simulink model "Full_Car_Model"  (R2023b)
settings: Solver=FixedStepAuto  StartTime=0.0  StopTime=t_end_sim  FixedStep=Ts_sim  RelTol=1e-3
values from neighbouring files (symbols this model uses):
  a_b_ref_sat = [ zeros(1,10) ... (first row only)    [A1_Init.m]    (also in C1_MonteCarloAnalysis.m)
  adaptive = 3    [A1_Init.m]    (also in C1_MonteCarloAnalysis.m = 1)
  data = A2_Full_car_model_parameters_4onBoard()    [A1_Init.m]    (also in C1_MonteCarloAnalysis.m)
  Ft_demand_F = [zeros(1,601) 200*ones(1,2400)]./data.R_F    [A1_Init.m]    (also in C1_MonteCarloAnalysis.m)
  Ft_demand_R = [zeros(1,(601-length(l_discr)))              200*ones(1,(2400+length(l_discr)))]./data.R_R    [A1_Init.m]    (also in C1_MonteCarloAnalysis.m)
  handmade_front = strcat(currentPath,'\Road_profiles\height_crg_files\','handmade_step_3cm_singlefunctions.crg')    [A1_Init.m]    (also in C1_MonteCarloAnalysis.m)
  handmade_mu_front = strcat(currentPath,'\Road_profiles\friction_crg_files\','handmade_fric_step_01_singlefunctions.crg')    [A1_Init.m]    (also in C1_MonteCarloAnalysis.m)
  handmade_mu_rear = handmade_mu_front    [A1_Init.m]    (also in C1_MonteCarloAnalysis.m)
  handmade_rear = handmade_front    [A1_Init.m]    (also in C1_MonteCarloAnalysis.m)
  LowLim_Q1 = -10    [A1_Init.m]    (also in C1_MonteCarloAnalysis.m)
  M = N    (= 10)    [A1_Init.m]    (also in C1_MonteCarloAnalysis.m)
  mu_distance = test_distance    [A1_Init.m]    (also in C1_MonteCarloAnalysis.m)
  mu_road = [ones(1,1001), 0.1*ones(1,2000)]    [A1_Init.m]    (also in C1_MonteCarloAnalysis.m)
  N = 10    [A1_Init.m]    (also in C1_MonteCarloAnalysis.m)
  N_iter = 3    [A1_Init.m]    (also in C1_MonteCarloAnalysis.m)
  omega_ini_F_L = x_u_dot_ini_F_L/data.R_F    [A1_Init.m]    (also in C1_MonteCarloAnalysis.m)
  omega_ini_F_R = x_u_dot_ini_R_R/data.R_F    [A1_Init.m]    (also in C1_MonteCarloAnalysis.m)
  omega_ini_R_L = x_u_dot_ini_R_L/data.R_R +2.483*1e-6    [A1_Init.m]    (also in C1_MonteCarloAnalysis.m)
  omega_ini_R_R = x_u_dot_ini_R_R/data.R_R+2.483*1e-6    [A1_Init.m]    (also in C1_MonteCarloAnalysis.m)
  passive = 2    [A1_Init.m]    (also in C1_MonteCarloAnalysis.m)
  Pitch = 0    [A1_Init.m]    (also in C1_MonteCarloAnalysis.m)
  Pitch_dot = 0    [A1_Init.m]    (also in C1_MonteCarloAnalysis.m)
  preview = 2    [A1_Init.m]    (also in C1_MonteCarloAnalysis.m)
  Q1 = 1e6    (= 1000000)    [A1_Init.m]    (also in C1_MonteCarloAnalysis.m)
  Q1_sat = 0    [A1_Init.m]    (also in C1_MonteCarloAnalysis.m)
  Q2 = 1e5    (= 100000)    [A1_Init.m]    (also in C1_MonteCarloAnalysis.m)
  QN1 = 0    [A1_Init.m]    (also in C1_MonteCarloAnalysis.m)
  QN2 = 0    [A1_Init.m]    (also in C1_MonteCarloAnalysis.m)
  R1 = 1e10    (= 10000000000)    [A1_Init.m]    (also in C1_MonteCarloAnalysis.m)
  r1_h0 = 0.99    [A1_Init.m]    (also in C1_MonteCarloAnalysis.m)
  r1_k = 1000    [A1_Init.m]    (also in C1_MonteCarloAnalysis.m)
  r1_max = 11    [A1_Init.m]    (also in C1_MonteCarloAnalysis.m)
  r1_min = -10    [A1_Init.m]    (also in C1_MonteCarloAnalysis.m)
  r2 = 2    [A1_Init.m]    (also in C1_MonteCarloAnalysis.m)
  R2 = 1e2    (= 100)    [A1_Init.m]    (also in C1_MonteCarloAnalysis.m)
  R2_rl = 2    [A1_Init.m]    (also in C1_MonteCarloAnalysis.m)
  road_profile = [zeros(1,801),ones(1,2200)*10*Step_selector]    [A1_Init.m]    (also in C1_MonteCarloAnalysis.m)
  T_distance = test_distance    [A1_Init.m]    (also in C1_MonteCarloAnalysis.m)
  T_hs_ini_F_L = 0    [A1_Init.m]    (also in C1_MonteCarloAnalysis.m)
  T_hs_ini_F_R = 0    [A1_Init.m]    (also in C1_MonteCarloAnalysis.m)
  T_hs_ini_R_L = 0    [A1_Init.m]    (also in C1_MonteCarloAnalysis.m)
  T_hs_ini_R_R = 0    [A1_Init.m]    (also in C1_MonteCarloAnalysis.m)
  test_distance = 0:0.01:30    [A1_Init.m]    (also in C1_MonteCarloAnalysis.m)
  theta_s_ini_F_L = 0    [A1_Init.m]    (also in C1_MonteCarloAnalysis.m)
  theta_s_ini_F_R = 0    [A1_Init.m]    (also in C1_MonteCarloAnalysis.m)
  theta_s_ini_R_L = 0    [A1_Init.m]    (also in C1_MonteCarloAnalysis.m)
  theta_s_ini_R_R = 0    [A1_Init.m]    (also in C1_MonteCarloAnalysis.m)
  theta_w_ini_F_L = -1.056*1e-2    (= -0.01056)    [A1_Init.m]    (also in C1_MonteCarloAnalysis.m)
  theta_w_ini_R_L = -1.056*1e-2    (= -0.01056)    [A1_Init.m]    (also in C1_MonteCarloAnalysis.m)
  Ts = 1e-3*[0 5 10 15 20 25 30 40 60 80 100]    [A1_Init.m]    (also in C1_MonteCarloAnalysis.m)
  w1_h0 = 0.0008    [A1_Init.m]    (also in C1_MonteCarloAnalysis.m)
  w1_k = 5000    [A1_Init.m]    (also in C1_MonteCarloAnalysis.m)
  w1_max = 9    [A1_Init.m]    (also in C1_MonteCarloAnalysis.m)
  w1_min = -10    [A1_Init.m]    (also in C1_MonteCarloAnalysis.m)
  w1_sat = 0.085    [A1_Init.m]    (also in C1_MonteCarloAnalysis.m)
  w2_h0 = 2    [A1_Init.m]    (also in C1_MonteCarloAnalysis.m)
  w2_inc = 0.05    [A1_Init.m]    (also in C1_MonteCarloAnalysis.m)
  w2_k = 10    [A1_Init.m]    (also in C1_MonteCarloAnalysis.m)
  w2_max = 5.3    [A1_Init.m]    (also in C1_MonteCarloAnalysis.m)
  w2_min = -10    [A1_Init.m]    (also in C1_MonteCarloAnalysis.m)
  Wmat_NMPC_init = [W(1,:) W(2,:) W(3,:) W(4,:)]    [A1_Init.m]    (also in C1_MonteCarloAnalysis.m)
  WNmat_NMPC_init = [WN(1,:) WN(2,:)]    [A1_Init.m]    (also in C1_MonteCarloAnalysis.m)
  X_0 = [z_b_dot_ini z_b_ini z_u_dot_ini_F_L z_u_ini_F_L x_b_dot_ini x_b_ini x_u_dot_ini_F_L x_u_ini_F_L          omega_ini_F_L theta_w_ini_F_L omega_ini_F_L theta_s_ini_F_L torque_ini_F_L]    [A1_Init.m]    (also in C1_MonteCarloAnalysis.m)
  x_b_dot_ini = speed_ini/3.6    (= 11.1111111111)    [A1_Init.m]    (also in C1_MonteCarloAnalysis.m)
  x_b_ini = data.b+pos_ini    [A1_Init.m]    (also in C1_MonteCarloAnalysis.m)
  x_u_dot_ini_F_L = speed_ini/3.6 - 1.125*1e-4    (= 11.1109986111)    [A1_Init.m]    (also in C1_MonteCarloAnalysis.m)
  x_u_dot_ini_F_R = speed_ini/3.6 - 1.125*1e-4    (= 11.1109986111)    [A1_Init.m]    (also in C1_MonteCarloAnalysis.m)
  x_u_dot_ini_R_L = speed_ini/3.6 - 1.125*1e-4    (= 11.1109986111)    [A1_Init.m]    (also in C1_MonteCarloAnalysis.m)
  x_u_dot_ini_R_R = speed_ini/3.6 - 1.125*1e-4    (= 11.1109986111)    [A1_Init.m]    (also in C1_MonteCarloAnalysis.m)
  x_u_ini_F_L = data.a+data.b+pos_ini    [A1_Init.m]    (also in C1_MonteCarloAnalysis.m)
  x_u_ini_F_R = data.a+data.b+pos_ini    [A1_Init.m]    (also in C1_MonteCarloAnalysis.m)
  x_u_ini_R_L = pos_ini    (= 0)    [A1_Init.m]    (also in C1_MonteCarloAnalysis.m)
  x_u_ini_R_R = pos_ini    (= 0)    [A1_Init.m]    (also in C1_MonteCarloAnalysis.m)
  z_b_dot_ini = 0    [A1_Init.m]    (also in C1_MonteCarloAnalysis.m)
  z_b_ini = 0    [A1_Init.m]    (also in C1_MonteCarloAnalysis.m)
  z_u_dot_ini_F_L = 0    [A1_Init.m]    (also in C1_MonteCarloAnalysis.m)
  z_u_dot_ini_F_R = 0    [A1_Init.m]    (also in C1_MonteCarloAnalysis.m)
  z_u_dot_ini_R_L = 0    [A1_Init.m]    (also in C1_MonteCarloAnalysis.m)
  z_u_dot_ini_R_R = 0    [A1_Init.m]    (also in C1_MonteCarloAnalysis.m)
  z_u_ini_F_L = 0    [A1_Init.m]    (also in C1_MonteCarloAnalysis.m)
  z_u_ini_F_R = 0    [A1_Init.m]    (also in C1_MonteCarloAnalysis.m)
  z_u_ini_R_L = 0    [A1_Init.m]    (also in C1_MonteCarloAnalysis.m)
  z_u_ini_R_R = 0    [A1_Init.m]    (also in C1_MonteCarloAnalysis.m)
undefined symbols (not defined in the file or in its folder): Delay_step, road_with_noise
libraries: mfswift_library x8, rllib x4, simulink x4
(part 3 of 7)

== system Full_Car_Model/CONTROLLER FRONT RIGHT/Weight matrixes ==
  x_u : Inport
  MATLAB Function : MATLAB Function  TreatAsAtomicUnit=on
  Q1 : Lookup_n-D  NumberOfTableDimensions=1  BreakpointsForDimension1=[0 1e6]  Table=[Q1 Q1]  InternalRulePriority=Speed  RndMeth=Simplest
  Q2 : Lookup_n-D  NumberOfTableDimensions=1  BreakpointsForDimension1=[0 1e6]  Table=[Q2 Q2]  InternalRulePriority=Speed  RndMeth=Simplest
  QN1 : Lookup_n-D  NumberOfTableDimensions=1  BreakpointsForDimension1=[0 1e6]  Table=[QN1 QN1]  InternalRulePriority=Speed  RndMeth=Simplest
  QN2 : Lookup_n-D  NumberOfTableDimensions=1  BreakpointsForDimension1=[0 1e6]  Table=[QN2 QN2]  InternalRulePriority=Speed  RndMeth=Simplest
  R1 : Lookup_n-D  NumberOfTableDimensions=1  BreakpointsForDimension1=[0 1e6]  Table=[R1 R1]  InternalRulePriority=Speed  RndMeth=Simplest
  R2 : Lookup_n-D  NumberOfTableDimensions=1  BreakpointsForDimension1=[0 1e6]  Table=[R2 R2]  InternalRulePriority=Speed  RndMeth=Simplest
  Scope : Scope
  Stage Cost Matrix : Outport
  Terminal Cost Matrix : Outport  Port=2
  wires:
  QN2/1 -> MATLAB Function/4(QN2)  "QN2"
  QN1/1 -> MATLAB Function/3(QN1)  "QN1"
  R2/1 -> MATLAB Function/6(R2)  "R2"
  R1/1 -> MATLAB Function/5(R1)  "R1"
  Q2/1 -> MATLAB Function/2(Q2)  "Q2"
  Q1/1 -> MATLAB Function/1(Q1)  "Q1"
  x_u/1 -> R2/1, R1/1, QN2/1, QN1/1, Q2/1, Q1/1
  MATLAB Function/2(WNmat_NMPC) -> Terminal Cost Matrix/1
  MATLAB Function/1(Wmat_NMPC) -> Stage Cost Matrix/1, Scope/1

== system Full_Car_Model/CONTROLLER REAR LEFT/RL_weights ==
  States : Inport
  Online Data : Inport  Port=2
  a_b_ref : Inport  Port=3
  Add : Sum  Inputs=+-
  Add1 : Sum  Inputs=+-
  Add2 : Sum  Inputs=+-
  Bus Selector : BusSelector  OutputSignals=Accelerations.x_b_ddot,Differentials.theta_s_dot_R_L,States.omega_R_L,States.slip_R_L,Traction_forces.Tm_R_L_req
  Control action R : Scope
  Demux : Demux  Commented=on  Outputs=3
  MATLAB Function : MATLAB Function  TreatAsAtomicUnit=on
  MATLAB Function3 : MATLAB Function  TreatAsAtomicUnit=on
  Memory1 : Memory  Commented=on  InheritSampleTime=on
  Memory2 : Memory  InheritSampleTime=on
  Memory4 : Memory  Commented=on  InheritSampleTime=on
  Memory5 : Memory  Commented=on  InheritSampleTime=on
  Mux : Mux  Commented=on  Inputs=3
  Mux6 : Mux  Inputs=5
  Policy : rllib/Policy  MATFile=blockAgentData_rear.mat  SimUsingCodegen=off
  Selector{,1..2,4..5} (5 alike) : Selector  InputPortWidth=1  IndexOptions=Select all  Indices=1  OutputSizes=1
  Subsystem2 : Subsystem
  To Workspace : ToWorkspace  VariableName=exponents_RL_RL  SaveFormat=Timeseries  SampleTime=-1
  Zero-Order Hold : ZeroOrderHold  SampleTime=0.001
  exponents : Outport
  tag scope: exp_RL_rear=global
  wires:
  Mux6/1 -> Policy/1
  Bus Selector/1 -> Add/1  "<x_b_ddot>"
  Add/1 -> Selector/1  "acc_error"
  Add1/1 -> Selector1/1  "delta_omega_error"
  Bus Selector/2 -> Add1/1  "<theta_s_dot_R_L>"
  Bus Selector/3 -> Add1/2  "<omega_R_L>"
  Bus Selector/4 -> Add2/2  "<slip_R_L>"
  Add2/1 -> Selector2/1  "slip_error"
  MATLAB Function3/1(h) -> Selector5/1  "r1"
  MATLAB Function/1(h) -> Selector4/1  "w1"
  Memory2/1 -> Zero-Order Hold/1, exponents/1, [exp_RL_rear], Control action R/1
  Selector/1 -> Mux6/1  "w1"
  Selector1/1 -> Mux6/2  "w1"
  Selector2/1 -> Mux6/3  "w1"
  Selector4/1 -> Mux6/4  "w1"
  Selector5/1 -> Mux6/5  "w1"
  States/1 -> Bus Selector/1
  a_b_ref/1 -> Add/2
  Policy/1 -> Memory2/1, Demux/1  "weights"
  Mux/1 -> ?
  Demux/1 -> Memory1/1
  Demux/3 -> Memory5/1
  Memory4/1 -> Mux/2
  Demux/2 -> Memory4/1
  Memory5/1 -> Mux/3
  Memory1/1 -> Mux/1
  Subsystem2/1(w_prev) -> MATLAB Function/1(w_prev)  "w_prev"
  Subsystem2/3(sigma_ref_act) -> Add2/1
  Subsystem2/2(mu_act_prev) -> MATLAB Function3/1(mu_prev)  "mu_act_prev"
  Online Data/1 -> Subsystem2/1(Online Data)
  Zero-Order Hold/1 -> To Workspace/1

== system Full_Car_Model/CONTROLLER REAR LEFT/ROAD PREVIEW ==
  F_t : Inport
  CAN : Inport  Port=2
  1-D Lookup Table : Lookup_n-D  NumberOfTableDimensions=1  BreakpointsForDimension1=[0.1:0.1:1]  Table=[0.005 0.01 0.016 0.02 0.025 0.03 0.04 0.05 0.055 0.06]  InternalRulePriority=Speed  RndMeth=Simplest
  1-D Lookup Table1 : Lookup_n-D  NumberOfTableDimensions=1  BreakpointsForDimension1=[0.1:0.1:1]  Table=[0.005 0.01 0.016 0.02 0.025 0.03 0.04 0.05 0.055 0.06]  InternalRulePriority=Speed  RndMeth=Simplest
  1-D Lookup Table2 : Lookup_n-D  NumberOfTableDimensions=1  BreakpointsForDimension1=mu_distance  Table=mu_road  InternalRulePriority=Speed  RndMeth=Simplest
  Bus Selector2 : BusSelector  OutputSignals=States.z_u_R_L
  Bus Selector3 : BusSelector  OutputSignals=States.x_u_R_L,States.x_u_dot_R_L,Traction_forces.Ft_F_req
  Constant : Constant
  Constant1 : Constant  Value=preview
  Constant2 : Constant
  Gain1 : Gain  Gain=data.R_R
  Multiply1 : Gain  Gain=data.R_F
  Multiply10 : Gain  Gain=1500/data.Tm_max
  Multiply12 : Gain  Gain=1500/data.Tm_max
  Multiport Switch2 : MultiPortSwitch  Inputs=2  SaturateOnIntegerOverflow=off  InputSameDT=off
  NO_ROAD_PREVIEW : MATLAB Function  TreatAsAtomicUnit=on
  Product : Product
  Product1 : Product
  ROAD PREVIEW : MATLAB Function  TreatAsAtomicUnit=on
  Time-based Road Preview : Subsystem
  To Workspace : ToWorkspace  VariableName=slip_ref_rear_sim  SaveFormat=Timeseries  SampleTime=-1
  To Workspace2 : ToWorkspace  VariableName=mu_rear_sim  SaveFormat=Timeseries  SampleTime=-1
  Online Data : Outport
  tag scope: mu_RL_LUT=global, slip_ref_R=global
  wires:
  CAN/1 -> Bus Selector2/1, Bus Selector3/1
  Multiport Switch2/1 -> Online Data/1
  Constant1/1 -> Multiport Switch2/1
  Bus Selector3/1 -> 1-D Lookup Table2/1, Time-based Road Preview/1(x_u)  "<x_u_R_L>"
  Bus Selector3/2 -> Time-based Road Preview/2(x_u_dot)  "<x_u_dot_R_L>"
  NO_ROAD_PREVIEW/1(OnlineData) -> Multiport Switch2/2  "Online Data"
  Time-based Road Preview/1(w) -> ROAD PREVIEW/1(w)
  Gain1/1 -> Multiply12/1, ROAD PREVIEW/3(Tm_req), NO_ROAD_PREVIEW/2(Tm_req)
  Bus Selector3/3 -> Product1/1  "<Ft_F_req>"
  Multiply1/1 -> Multiply10/1
  Bus Selector2/1 -> NO_ROAD_PREVIEW/1(w)  "<z_u_R_L>"
  1-D Lookup Table/1 -> ROAD PREVIEW/8(sigma_ref)
  Time-based Road Preview/2(beta_y) -> ROAD PREVIEW/2(beta_y)
  Product/1 -> NO_ROAD_PREVIEW/3(Tm_req_R2), ROAD PREVIEW/4(Tm_req_R2)
  Multiply12/1 -> Product/1
  ROAD PREVIEW/1(OnlineData) -> Multiport Switch2/3  "Online Data"
  Time-based Road Preview/3(mu_prev) -> 1-D Lookup Table/1, ROAD PREVIEW/7(mu_act)
  1-D Lookup Table2/1 -> 1-D Lookup Table1/1, NO_ROAD_PREVIEW/6(mu_act), [mu_RL_LUT], To Workspace2/1  "mu_R_L"
  1-D Lookup Table1/1 -> [slip_ref_R], To Workspace/1, NO_ROAD_PREVIEW/7(sigma_ref)
  [mu_RL_LUT] -> Product/2
  Product1/1 -> Multiply1/1
  [mu_FL_LUT] -> Product1/2
  F_t/1 -> Gain1/1
  Multiply10/1 -> ROAD PREVIEW/6(Tm_req_F_R), NO_ROAD_PREVIEW/4(Tm_req_F_L), NO_ROAD_PREVIEW/5(Tm_req_F_R), ROAD PREVIEW/5(Tm_req_F_L)

== system Full_Car_Model/CONTROLLER REAR LEFT/Reference acceleration ==
  Ft : Inport
  x_b_dot : Inport  Port=2
  Ft2 : Inport  Port=3
  2-D Lookup Table : Lookup_n-D  BreakpointsForDimension1=[0:50:350]  BreakpointsForDimension2=[0.1:0.1:1]  Table=a_b_ref_sat  InternalRulePriority=Speed  RndMeth=Simplest
      settings: InputPortMap=u0,u1
  2-D Lookup Table1 : Lookup_n-D  BreakpointsForDimension1=[0:50:350]  BreakpointsForDimension2=[0.1:0.1:1]  Table=a_b_ref_sat  InternalRulePriority=Speed  RndMeth=Simplest
      settings: InputPortMap=u0,u1
  Add : Sum
  Add1 : Sum
  Constant : Constant  Value=-Inf
  Gain : Gain  Gain=0.5
  Gain1 : Gain  Gain=0.5
  Gain2 : Gain  Gain=data.R_R
  Gain3 : Gain  Gain=data.R_F
  Saturation Dynamic : simulink/Discontinuities/Saturation Dynamic  OutMin=[]  OutMax=[]  OutDataTypeStr=Inherit: Same as second input  OutDataType=fixdt(1, 16)  OutScaling=2^-10  DoSatur=off
  a_b_ref : MATLAB Function  TreatAsAtomicUnit=on
  a_ref : Outport
  wires:
  Ft/1 -> Add/1, Gain2/1  "Ft"
  Gain2/1 -> 2-D Lookup Table/1
  Constant/1 -> Saturation Dynamic/3
  Saturation Dynamic/1 -> a_ref/1  "a_b_ref"
  x_b_dot/1 -> a_b_ref/2(vCar_k)  "x_b_dot"
  a_b_ref/1(a_b_ref) -> Saturation Dynamic/2
  Add/1 -> a_b_ref/1(Ft)
  Ft2/1 -> Gain3/1, Add/2  "Ft2"
  Add1/1 -> Saturation Dynamic/1
  Gain3/1 -> 2-D Lookup Table1/1
  [mu_RL_LUT] -> 2-D Lookup Table/2
  [mu_FL_LUT] -> 2-D Lookup Table1/2
  2-D Lookup Table1/1 -> Gain1/1
  2-D Lookup Table/1 -> Gain/1
  Gain/1 -> Add1/1
  Gain1/1 -> Add1/2

== system Full_Car_Model/CONTROLLER REAR LEFT/Rule based ==
  Online Data : Inport
  BUS : Inport  Port=2
  Flag : Subsystem
  Gain4 : Gain  Gain=data.R_R
  MATLAB Function : MATLAB Function  TreatAsAtomicUnit=on
  MATLAB Function2 : MATLAB Function  TreatAsAtomicUnit=on
  MATLAB Function3 : MATLAB Function  TreatAsAtomicUnit=on
  Min : MinMax  Inputs=2
  Mux : Mux  Inputs=3
  Product : Product
  Selector : Selector  NumberOfDimensions=2  InputPortWidth=1  IndexOptions=Index vector (dialog),Select all  Indices=1,1  OutputSizes=1,1
  Subsystem : Subsystem
  To Workspace9 : ToWorkspace  VariableName=exponents_RL_RB  SaveFormat=Timeseries  SampleTime=-1
  Zero-Order Hold : ZeroOrderHold  SampleTime=0.001
  memory : Subsystem
  exponents : Outport
  tag scope: exp_RB_rear=global
  wires:
  Min/1 -> MATLAB Function/2(mu)
  [mu_FL_LUT] -> Min/1
  MATLAB Function3/1(W) -> Mux/3  "r1"
  Subsystem/1(w_prev) -> MATLAB Function/1(w_prev)  "w_prev"
  Selector/1 -> Min/2, Product/1, MATLAB Function2/2(mu)
  Gain4/1 -> memory/1(In1)
  memory/1(Out1) -> MATLAB Function2/1(dT_req)
  [Ft_req_R] -> Product/2
  Online Data/1 -> Subsystem/1(Online Data)
  MATLAB Function2/1(W) -> Mux/2  "w2"
  MATLAB Function/1(W) -> Mux/1  "w1"
  Mux/1 -> exponents/1, [exp_RB_rear], Zero-Order Hold/1
  Zero-Order Hold/1 -> To Workspace9/1
  Product/1 -> Gain4/1
  Flag/1(Flag) -> MATLAB Function3/1(flag)
  Subsystem/2(mu_act_prev) -> Flag/2(mu_prev), MATLAB Function3/2(mu_prev), Selector/1  "mu_act_prev"
  BUS/1 -> Flag/1(Measurement data)

== system Full_Car_Model/CONTROLLER REAR LEFT/Subsystem1 ==
  exponents : Inport
  Constant : Constant  Value=R2_rl
  Constant1 : Constant  Value=0
  Demux : Demux  Outputs=3
  Exp{,1..3} (4 alike) : Math  Operator=10^u
  MATLAB Function : MATLAB Function  TreatAsAtomicUnit=on
  MATLAB Function1 : MATLAB Function  TreatAsAtomicUnit=on
  MATLAB Function2 : MATLAB Function  TreatAsAtomicUnit=on
  Min : MinMax  Inputs=2
  stage cost matrix : Outport
  terminal cost matrix : Outport  Port=2
  wires:
  MATLAB Function/1(Wmat_NMPC) -> stage cost matrix/1
  MATLAB Function1/1(WNmat_NMPC) -> terminal cost matrix/1
  exponents/1 -> Demux/1
  Demux/1 -> MATLAB Function2/1(Q1)
  Demux/2 -> Exp1/1
  Demux/3 -> Exp2/1
  Exp/1 -> MATLAB Function/1(Q1)
  Exp1/1 -> MATLAB Function/2(Q2)
  Exp2/1 -> MATLAB Function/3(R1)
  Constant/1 -> Exp3/1
  Exp3/1 -> MATLAB Function/4(R2)
  Constant1/1 -> MATLAB Function1/2(QN2), MATLAB Function1/1(QN1)
  [mu_FL_LUT] -> Min/1
  [mu_RL_LUT] -> Min/2
  Min/1 -> MATLAB Function2/2(mu)
  MATLAB Function2/1(Q1_out) -> Exp/1

== system Full_Car_Model/CONTROLLER REAR LEFT/Subsystem2 ==
  exponents : Inport
  Constant : Constant  Value=r2
  Constant1 : Constant  Value=0
  Demux : Demux  Outputs=3
  Exp{,1..4} (5 alike) : Math  Operator=10^u
  MATLAB Function : MATLAB Function  TreatAsAtomicUnit=on
  MATLAB Function1 : MATLAB Function  TreatAsAtomicUnit=on
  stage cost matrix : Outport
  terminal cost matrix : Outport  Port=2
  wires:
  MATLAB Function/1(Wmat_NMPC) -> stage cost matrix/1
  MATLAB Function1/1(WNmat_NMPC) -> terminal cost matrix/1
  exponents/1 -> Demux/1
  Demux/1 -> Exp/1
  Demux/2 -> Exp1/1
  Demux/3 -> Exp2/1
  Exp/1 -> MATLAB Function/1(Q1)
  Exp1/1 -> MATLAB Function/2(Q2)
  Exp2/1 -> MATLAB Function/3(R1)
  Constant/1 -> Exp3/1
  Exp3/1 -> MATLAB Function/4(R2)
  Constant1/1 -> Exp4/1
  Exp4/1 -> MATLAB Function1/2(QN2), MATLAB Function1/1(QN1)

== system Full_Car_Model/CONTROLLER REAR LEFT/Weight matrixes ==
  x_u : Inport
  MATLAB Function : MATLAB Function  TreatAsAtomicUnit=on
  Q1 : Lookup_n-D  NumberOfTableDimensions=1  BreakpointsForDimension1=[0 1e6]  Table=[Q1 Q1]  InternalRulePriority=Speed  RndMeth=Simplest
  Q2 : Lookup_n-D  NumberOfTableDimensions=1  BreakpointsForDimension1=[0 1e6]  Table=[Q2 Q2]  InternalRulePriority=Speed  RndMeth=Simplest
  QN1 : Lookup_n-D  NumberOfTableDimensions=1  BreakpointsForDimension1=[0 1e6]  Table=[QN1 QN1]  InternalRulePriority=Speed  RndMeth=Simplest
  QN2 : Lookup_n-D  NumberOfTableDimensions=1  BreakpointsForDimension1=[0 1e6]  Table=[QN2 QN2]  InternalRulePriority=Speed  RndMeth=Simplest
  R1 : Lookup_n-D  NumberOfTableDimensions=1  BreakpointsForDimension1=[0 1e6]  Table=[R1 R1]  InternalRulePriority=Speed  RndMeth=Simplest
  R2 : Lookup_n-D  NumberOfTableDimensions=1  BreakpointsForDimension1=[0 1e6]  Table=[R2 R2]  InternalRulePriority=Speed  RndMeth=Simplest
  Scope : Scope
  Stage Cost Matrix : Outport
  Terminal Cost Matrix : Outport  Port=2
  wires:
  QN2/1 -> MATLAB Function/4(QN2)  "QN2"
  QN1/1 -> MATLAB Function/3(QN1)  "QN1"
  R2/1 -> MATLAB Function/6(R2)  "R2"
  R1/1 -> MATLAB Function/5(R1)  "R1"
  Q2/1 -> MATLAB Function/2(Q2)  "Q2"
  Q1/1 -> MATLAB Function/1(Q1)  "Q1"
  x_u/1 -> R2/1, R1/1, QN2/1, QN1/1, Q2/1, Q1/1
  MATLAB Function/2(WNmat_NMPC) -> Terminal Cost Matrix/1
  MATLAB Function/1(Wmat_NMPC) -> Stage Cost Matrix/1, Scope/1

== system Full_Car_Model/CONTROLLER REAR RIGHT/RL_weights ==
  States : Inport
  Online Data : Inport  Port=2
  a_b_ref : Inport  Port=3
  Add : Sum  Inputs=+-
  Add1 : Sum  Inputs=+-
  Add2 : Sum  Inputs=+-
  Bus Selector : BusSelector  OutputSignals=Accelerations.x_b_ddot,Differentials.theta_s_dot_R_R,States.omega_R_R,States.slip_R_R
  Control action : Scope
  Demux : Demux  Commented=on  Outputs=3
  MATLAB Function : MATLAB Function  TreatAsAtomicUnit=on
  MATLAB Function3 : MATLAB Function  TreatAsAtomicUnit=on
  Memory1 : Memory  Commented=on  InheritSampleTime=on
  Memory2 : Memory  InheritSampleTime=on
  Memory4 : Memory  Commented=on  InheritSampleTime=on
  Memory5 : Memory  Commented=on  InheritSampleTime=on
  Mux : Mux  Commented=on  Inputs=3
  Mux6 : Mux  Inputs=5
  Policy : rllib/Policy  MATFile=blockAgentData_rear.mat  SimUsingCodegen=off
  Selector{,1..2,4..5} (5 alike) : Selector  InputPortWidth=1  IndexOptions=Select all  Indices=1  OutputSizes=1
  Subsystem2 : Subsystem
  exponents : Outport
  wires:
  Mux6/1 -> Policy/1
  Bus Selector/1 -> Add/1  "<x_b_ddot>"
  Add/1 -> Selector/1  "acc_error"
  Add1/1 -> Selector1/1  "delta_omega_error"
  Bus Selector/2 -> Add1/1  "<theta_s_dot_R_R>"
  Bus Selector/3 -> Add1/2  "<omega_R_R>"
  Bus Selector/4 -> Add2/2  "<slip_R_R>"
  Add2/1 -> Selector2/1  "slip_error"
  Memory2/1 -> Control action/1, exponents/1
  Selector/1 -> Mux6/1  "w1"
  Selector1/1 -> Mux6/2  "w1"
  Selector2/1 -> Mux6/3  "w1"
  Selector4/1 -> Mux6/4  "w1"
  Selector5/1 -> Mux6/5  "w1"
  States/1 -> Bus Selector/1
  a_b_ref/1 -> Add/2
  Online Data/1 -> Subsystem2/1(Online Data)
  Mux/1 -> ?
  Demux/1 -> Memory1/1
  Policy/1 -> Memory2/1, Demux/1  "weights"
  Demux/3 -> Memory5/1
  Memory4/1 -> Mux/2
  Demux/2 -> Memory4/1
  Memory5/1 -> Mux/3
  Memory1/1 -> Mux/1
  Subsystem2/1(w_prev) -> MATLAB Function/1(w_prev)  "w_prev"
  Subsystem2/3(sigma_ref_act) -> Add2/1
  Subsystem2/2(mu_act_prev) -> MATLAB Function3/1(mu_prev)  "mu_act_prev"
  MATLAB Function/1(h) -> Selector4/1  "w1"
  MATLAB Function3/1(h) -> Selector5/1  "r1"

== system Full_Car_Model/CONTROLLER REAR RIGHT/ROAD PREVIEW ==
  F_t : Inport
  CAN : Inport  Port=2
  1-D Lookup Table : Lookup_n-D  NumberOfTableDimensions=1  BreakpointsForDimension1=[0.1:0.1:1]  Table=[0.005 0.01 0.016 0.02 0.025 0.03 0.04 0.05 0.055 0.06]  InternalRulePriority=Speed  RndMeth=Simplest
  1-D Lookup Table1 : Lookup_n-D  NumberOfTableDimensions=1  BreakpointsForDimension1=[0.1:0.1:1]  Table=[0.005 0.01 0.016 0.02 0.025 0.03 0.04 0.05 0.055 0.06]  InternalRulePriority=Speed  RndMeth=Simplest
  1-D Lookup Table2 : Lookup_n-D  NumberOfTableDimensions=1  BreakpointsForDimension1=mu_distance  Table=mu_road  InternalRulePriority=Speed  RndMeth=Simplest
  Bus Selector2 : BusSelector  OutputSignals=States.z_u_R_R
  Bus Selector3 : BusSelector  OutputSignals=States.x_u_R_R,States.x_u_dot_R_R,Traction_forces.Ft_F_req
  Constant : Constant
  Constant1 : Constant  Value=preview
  Constant2 : Constant
  Gain3 : Gain  Gain=data.R_R
  Multiply4 : Gain  Gain=data.R_F
  Multiply5 : Gain  Gain=1500/data.Tm_max
  Multiply6 : Gain  Gain=1500/data.Tm_max
  Multiport Switch2 : MultiPortSwitch  Inputs=2  SaturateOnIntegerOverflow=off  InputSameDT=off
  NO_ROAD_PREVIEW : MATLAB Function  TreatAsAtomicUnit=on
  Product2 : Product
  Product3 : Product
  ROAD PREVIEW : MATLAB Function  TreatAsAtomicUnit=on
  Time-based Road Preview : Subsystem
  Online Data : Outport
  tag scope: mu_RR_LUT=global
  wires:
  1-D Lookup Table1/1 -> NO_ROAD_PREVIEW/7(sigma_ref)
  Time-based Road Preview/3(mu_prev) -> 1-D Lookup Table/1, ROAD PREVIEW/7(mu_act)
  Product2/1 -> NO_ROAD_PREVIEW/3(Tm_req_R2), ROAD PREVIEW/4(Tm_req_R2)
  CAN/1 -> Bus Selector2/1, Bus Selector3/1
  Multiport Switch2/1 -> Online Data/1
  Bus Selector2/1 -> NO_ROAD_PREVIEW/1(w)  "<z_u_R_R>"
  Time-based Road Preview/1(w) -> ROAD PREVIEW/1(w)
  Time-based Road Preview/2(beta_y) -> ROAD PREVIEW/2(beta_y)
  Multiply5/1 -> ROAD PREVIEW/6(Tm_req_F_R), NO_ROAD_PREVIEW/4(Tm_req_F_L), NO_ROAD_PREVIEW/5(Tm_req_F_R), ROAD PREVIEW/5(Tm_req_F_L)
  1-D Lookup Table/1 -> ROAD PREVIEW/8(sigma_ref)
  ROAD PREVIEW/1(OnlineData) -> Multiport Switch2/3  "Online Data"
  Bus Selector3/1 -> 1-D Lookup Table2/1, Time-based Road Preview/1(x_u)  "<x_u_R_R>"
  Bus Selector3/2 -> Time-based Road Preview/2(x_u_dot)  "<x_u_dot_R_R>"
  NO_ROAD_PREVIEW/1(OnlineData) -> Multiport Switch2/2  "Online Data"
  Constant1/1 -> Multiport Switch2/1
  1-D Lookup Table2/1 -> [mu_RR_LUT], 1-D Lookup Table1/1, NO_ROAD_PREVIEW/6(mu_act)  "mu_R_R"
  Gain3/1 -> ROAD PREVIEW/3(Tm_req), Multiply6/1, NO_ROAD_PREVIEW/2(Tm_req)
  Bus Selector3/3 -> Product3/1  "<Ft_F_req>"
  [mu_RL_LUT] -> Product2/2
  [mu_FL_LUT] -> Product3/2
  Multiply6/1 -> Product2/1
  Product3/1 -> Multiply4/1
  F_t/1 -> Gain3/1
  Multiply4/1 -> Multiply5/1

== system Full_Car_Model/CONTROLLER REAR RIGHT/Reference acceleration ==
  Ft : Inport
  x_b_dot : Inport  Port=2
  Ft2 : Inport  Port=3
  2-D Lookup Table : Lookup_n-D  BreakpointsForDimension1=[0:50:350]  BreakpointsForDimension2=[0.1:0.1:1]  Table=a_b_ref_sat  InternalRulePriority=Speed  RndMeth=Simplest
      settings: InputPortMap=u0,u1
  2-D Lookup Table1 : Lookup_n-D  BreakpointsForDimension1=[0:50:350]  BreakpointsForDimension2=[0.1:0.1:1]  Table=a_b_ref_sat  InternalRulePriority=Speed  RndMeth=Simplest
      settings: InputPortMap=u0,u1
  Add : Sum
  Add1 : Sum
  Constant : Constant  Value=-Inf
  Gain : Gain  Gain=0.5
  Gain1 : Gain  Gain=0.5
  Gain2 : Gain  Gain=data.R_R
  Gain3 : Gain  Gain=data.R_F
  Saturation Dynamic : simulink/Discontinuities/Saturation Dynamic  OutMin=[]  OutMax=[]  OutDataTypeStr=Inherit: Same as second input  OutDataType=fixdt(1, 16)  OutScaling=2^-10  DoSatur=off
  a_b_ref : MATLAB Function  TreatAsAtomicUnit=on
  a_ref : Outport
  wires:
  Ft/1 -> Add/1, Gain2/1  "Ft"
  Gain2/1 -> 2-D Lookup Table/1
  Constant/1 -> Saturation Dynamic/3
  Saturation Dynamic/1 -> a_ref/1  "a_b_ref"
  x_b_dot/1 -> a_b_ref/2(vCar_k)  "x_b_dot"
  a_b_ref/1(a_b_ref) -> Saturation Dynamic/2
  Add/1 -> a_b_ref/1(Ft)
  Ft2/1 -> Gain3/1, Add/2  "Ft2"
  Add1/1 -> Saturation Dynamic/1
  Gain3/1 -> 2-D Lookup Table1/1
  [mu_RL_LUT] -> 2-D Lookup Table/2
  [mu_FL_LUT] -> 2-D Lookup Table1/2
  2-D Lookup Table1/1 -> Gain1/1
  2-D Lookup Table/1 -> Gain/1
  Gain/1 -> Add1/1
  Gain1/1 -> Add1/2

== system Full_Car_Model/CONTROLLER REAR RIGHT/Rule based ==
  Online Data : Inport
  BUS : Inport  Port=2
  Flag : Subsystem
  Gain4 : Gain  Gain=data.R_R
  MATLAB Function : MATLAB Function  TreatAsAtomicUnit=on
  MATLAB Function2 : MATLAB Function  TreatAsAtomicUnit=on
  MATLAB Function3 : MATLAB Function  TreatAsAtomicUnit=on
  Min : MinMax  Inputs=2
  Mux : Mux  Inputs=3
  Product : Product
  Selector : Selector  NumberOfDimensions=2  InputPortWidth=1  IndexOptions=Index vector (dialog),Select all  Indices=1,1  OutputSizes=1,1
  Subsystem : Subsystem
  memory : Subsystem
  exponents : Outport
  wires:
  Min/1 -> MATLAB Function/2(mu)
  [mu_FL_LUT] -> Min/1
  MATLAB Function3/1(W) -> Mux/3  "r1"
  Subsystem/1(w_prev) -> MATLAB Function/1(w_prev)  "w_prev"
  Selector/1 -> Min/2, Product/1, MATLAB Function2/2(mu)
  Gain4/1 -> memory/1(In1)
  memory/1(Out1) -> MATLAB Function2/1(dT_req)
  [Ft_req_R] -> Product/2
  Online Data/1 -> Subsystem/1(Online Data)
  MATLAB Function2/1(W) -> Mux/2  "w2"
  MATLAB Function/1(W) -> Mux/1  "w1"
  Mux/1 -> exponents/1
  Product/1 -> Gain4/1
  Subsystem/2(mu_act_prev) -> Flag/2(mu_prev), MATLAB Function3/2(mu_prev), Selector/1  "mu_act_prev"
  Flag/1(Flag) -> MATLAB Function3/1(flag)
  BUS/1 -> Flag/1(Measurement data)

== system Full_Car_Model/CONTROLLER REAR RIGHT/Subsystem1 ==
  exponents : Inport
  Constant : Constant  Value=R2_rl
  Constant1 : Constant  Value=0
  Demux : Demux  Outputs=3
  Exp{,1..3} (4 alike) : Math  Operator=10^u
  MATLAB Function : MATLAB Function  TreatAsAtomicUnit=on
  MATLAB Function1 : MATLAB Function  TreatAsAtomicUnit=on
  MATLAB Function2 : MATLAB Function  TreatAsAtomicUnit=on
  Min : MinMax  Inputs=2
  stage cost matrix : Outport
  terminal cost matrix : Outport  Port=2
  wires:
  MATLAB Function/1(Wmat_NMPC) -> stage cost matrix/1
  MATLAB Function1/1(WNmat_NMPC) -> terminal cost matrix/1
  exponents/1 -> Demux/1
  Demux/1 -> MATLAB Function2/1(Q1)
  Demux/2 -> Exp1/1
  Demux/3 -> Exp2/1
  Exp/1 -> MATLAB Function/1(Q1)
  Exp1/1 -> MATLAB Function/2(Q2)
  Exp2/1 -> MATLAB Function/3(R1)
  Constant/1 -> Exp3/1
  Exp3/1 -> MATLAB Function/4(R2)
  Constant1/1 -> MATLAB Function1/2(QN2), MATLAB Function1/1(QN1)
  [mu_FL_LUT] -> Min/1
  [mu_RL_LUT] -> Min/2
  Min/1 -> MATLAB Function2/2(mu)
  MATLAB Function2/1(Q1_out) -> Exp/1

== system Full_Car_Model/CONTROLLER REAR RIGHT/Subsystem2 ==
  exponents : Inport
  Constant : Constant  Value=r2
  Constant1 : Constant  Value=0
  Demux : Demux  Outputs=3
  Exp{,1..4} (5 alike) : Math  Operator=10^u
  MATLAB Function : MATLAB Function  TreatAsAtomicUnit=on
  MATLAB Function1 : MATLAB Function  TreatAsAtomicUnit=on
  stage cost matrix : Outport
  terminal cost matrix : Outport  Port=2
  wires:
  MATLAB Function/1(Wmat_NMPC) -> stage cost matrix/1
  MATLAB Function1/1(WNmat_NMPC) -> terminal cost matrix/1
  exponents/1 -> Demux/1
  Demux/1 -> Exp/1
  Demux/2 -> Exp1/1
  Demux/3 -> Exp2/1
  Exp/1 -> MATLAB Function/1(Q1)
  Exp1/1 -> MATLAB Function/2(Q2)
  Exp2/1 -> MATLAB Function/3(R1)
  Constant/1 -> Exp3/1
  Exp3/1 -> MATLAB Function/4(R2)
  Constant1/1 -> Exp4/1
  Exp4/1 -> MATLAB Function1/2(QN2), MATLAB Function1/1(QN1)

== system Full_Car_Model/CONTROLLER REAR RIGHT/Weight matrixes ==
  x_u : Inport
  MATLAB Function : MATLAB Function  TreatAsAtomicUnit=on
  Q1 : Lookup_n-D  NumberOfTableDimensions=1  BreakpointsForDimension1=[0 1e6]  Table=[Q1 Q1]  InternalRulePriority=Speed  RndMeth=Simplest
  Q2 : Lookup_n-D  NumberOfTableDimensions=1  BreakpointsForDimension1=[0 1e6]  Table=[Q2 Q2]  InternalRulePriority=Speed  RndMeth=Simplest
  QN1 : Lookup_n-D  NumberOfTableDimensions=1  BreakpointsForDimension1=[0 1e6]  Table=[QN1 QN1]  InternalRulePriority=Speed  RndMeth=Simplest
  QN2 : Lookup_n-D  NumberOfTableDimensions=1  BreakpointsForDimension1=[0 1e6]  Table=[QN2 QN2]  InternalRulePriority=Speed  RndMeth=Simplest
  R1 : Lookup_n-D  NumberOfTableDimensions=1  BreakpointsForDimension1=[0 1e6]  Table=[R1 R1]  InternalRulePriority=Speed  RndMeth=Simplest
  R2 : Lookup_n-D  NumberOfTableDimensions=1  BreakpointsForDimension1=[0 1e6]  Table=[R2 R2]  InternalRulePriority=Speed  RndMeth=Simplest
  Scope : Scope
  Stage Cost Matrix : Outport
  Terminal Cost Matrix : Outport  Port=2
  wires:
  QN2/1 -> MATLAB Function/4(QN2)  "QN2"
  QN1/1 -> MATLAB Function/3(QN1)  "QN1"
  R2/1 -> MATLAB Function/6(R2)  "R2"
  R1/1 -> MATLAB Function/5(R1)  "R1"
  Q2/1 -> MATLAB Function/2(Q2)  "Q2"
  Q1/1 -> MATLAB Function/1(Q1)  "Q1"
  x_u/1 -> R2/1, R1/1, QN2/1, QN1/1, Q2/1, Q1/1
  MATLAB Function/2(WNmat_NMPC) -> Terminal Cost Matrix/1
  MATLAB Function/1(Wmat_NMPC) -> Stage Cost Matrix/1, Scope/1

== system Full_Car_Model/NMPC Internal model FL/Time-based Road Preview ==
  x_u : Inport
  Delay1 : Delay  Commented=on  DelayLength=Delay_step
  Gain1 : Gain  Gain=1e-3
  Goto5 : Goto  Commented=on  GotoTag=beta_y_env_F_L  TagVisibility=global
  Goto6 : Goto  Commented=on  GotoTag=w_env_F_L  TagVisibility=global
  MATLAB Function1 : MATLAB Function  TreatAsAtomicUnit=on
  MATLAB Function4 : MATLAB Function  TreatAsAtomicUnit=on
  MATLAB Function5 : MATLAB Function  TreatAsAtomicUnit=on
  Scope : Scope
  Z_road with noise2 : Lookup_n-D  Commented=on  NumberOfTableDimensions=1  BreakpointsForDimension1=test_distance  Table=road_with_noise  InterpMethod=Flat  InternalRulePriority=Speed  RndMeth=Simplest
  Z_road1 : Lookup_n-D  NumberOfTableDimensions=1  BreakpointsForDimension1=test_distance  Table=road_profile  InterpMethod=Flat  InternalRulePriority=Speed  RndMeth=Simplest
  w : Outport
  beta_y : Outport  Port=2
  wires:
  x_u/1 -> MATLAB Function5/1(X)
  MATLAB Function5/1(x_road) -> Z_road1/1
  Z_road1/1 -> Gain1/1
  MATLAB Function4/2(beta_y) -> Goto5/1, beta_y/1
  MATLAB Function1/1(Z_ef) -> MATLAB Function4/1(Z_ef)
  MATLAB Function1/2(Z_er) -> MATLAB Function4/2(Z_er)
  MATLAB Function4/1(w) -> Scope/1, w/1, Goto6/1  "w"
  Gain1/1 -> MATLAB Function1/1(z_road)

== system Full_Car_Model/PLANT MODEL WITH MF-SWIFT/4 ON-BOARD POWERTRAIN - FRONT ==
  T_m_L : Inport
  T_m_R : Inport  Port=2
  theta_w_L : Inport  Port=3
  omega_w_L : Inport  Port=4
  theta_w_R : Inport  Port=5
  omega_w_R : Inport  Port=6
  DIFFERENTIAL_L : Subsystem
  DIFFERENTIAL_R : Subsystem
  Integrator1 : Integrator  InitialCondition=theta_s_ini_F_L
  Integrator2 : Integrator  InitialCondition=omega_ini_F_L
  Integrator3 : Integrator  InitialCondition=theta_s_ini_F_R
  Integrator6 : Integrator  InitialCondition=omega_ini_F_R
  LEFT HALF SHAFT TORQUES WITH BACKLASH : Subsystem
  Memory : Memory  InitialCondition=T_hs_ini_F_L
  Memory1 : Memory  InitialCondition=T_hs_ini_F_R
  RIGHT HALF SHAFT TORQUES WITH BACKLASH : Subsystem
  SHAFT EQUATIONS : MATLAB Function  TreatAsAtomicUnit=on
  To Workspace : ToWorkspace  VariableName=Tm_FL_sim  SaveFormat=Timeseries  SampleTime=-1
  To Workspace1 : ToWorkspace  VariableName=Tm_FR_sim  SaveFormat=Timeseries  SampleTime=-1
  T_hs_L : Outport
  T_hs_R : Outport  Port=2
  tag scope: Tm_F_L=global, Tm_F_R=global, theta_s_F_L=global, theta_s_F_R=global, theta_s_ddot_F_L=global, theta_s_ddot_F_R=global, theta_s_dot_F_L=global, theta_s_dot_F_R=global
  wires:
  Integrator6/1 -> [theta_s_dot_F_R], Integrator3/1, RIGHT HALF SHAFT TORQUES WITH BACKLASH/1(omega_s)  "theta_s_dot_R"
  Integrator2/1 -> [theta_s_dot_F_L], Integrator1/1, LEFT HALF SHAFT TORQUES WITH BACKLASH/1(omega_s)  "theta_s_dot_L"
  Memory1/1 -> SHAFT EQUATIONS/4(T_hs_R)
  Integrator3/1 -> [theta_s_F_R], RIGHT HALF SHAFT TORQUES WITH BACKLASH/2(theta_s)  "theta_s_R"
  theta_w_R/1 -> RIGHT HALF SHAFT TORQUES WITH BACKLASH/3(theta_w)
  omega_w_L/1 -> LEFT HALF SHAFT TORQUES WITH BACKLASH/4(omega_w)
  omega_w_R/1 -> RIGHT HALF SHAFT TORQUES WITH BACKLASH/4(omega_w)
  RIGHT HALF SHAFT TORQUES WITH BACKLASH/1(T_hs) -> T_hs_R/1, Memory1/1  "T_hs_R"
  DIFFERENTIAL_L/1(T_t) -> SHAFT EQUATIONS/1(T_t_L)
  theta_w_L/1 -> LEFT HALF SHAFT TORQUES WITH BACKLASH/3(theta_w)
  Integrator1/1 -> [theta_s_F_L], LEFT HALF SHAFT TORQUES WITH BACKLASH/2(theta_s)  "theta_s_L"
  LEFT HALF SHAFT TORQUES WITH BACKLASH/1(T_hs) -> Memory/1, T_hs_L/1  "T_hs_L"
  Memory/1 -> SHAFT EQUATIONS/2(T_hs_L)
  DIFFERENTIAL_R/1(T_t) -> SHAFT EQUATIONS/3(T_t_R)
  T_m_R/1 -> [Tm_F_R], To Workspace1/1, DIFFERENTIAL_R/1(T_dm)
  T_m_L/1 -> DIFFERENTIAL_L/1(T_dm), [Tm_F_L], To Workspace/1
  SHAFT EQUATIONS/2(theta_s_ddot_R) -> [theta_s_ddot_F_R], Integrator6/1
  SHAFT EQUATIONS/1(theta_s_ddot_L) -> [theta_s_ddot_F_L], Integrator2/1

== system Full_Car_Model/PLANT MODEL WITH MF-SWIFT/4 ON-BOARD POWERTRAIN - REAR ==
  T_m_L : Inport
  T_m_R : Inport  Port=2
  theta_w_L : Inport  Port=3
  omega_w_L : Inport  Port=4
  theta_w_R : Inport  Port=5
  omega_w_R : Inport  Port=6
  DIFFERENTIAL_L : Subsystem
  DIFFERENTIAL_R : Subsystem
  Integrator1 : Integrator  InitialCondition=theta_s_ini_R_L
  Integrator3 : Integrator  InitialCondition=theta_s_ini_R_R
  Integrator4 : Integrator  InitialCondition=omega_ini_R_L
  Integrator5 : Integrator  InitialCondition=omega_ini_R_R
  LEFT HALF SHAFT TORQUES WITH BACKLASH : Subsystem
  Memory : Memory  InitialCondition=T_hs_ini_R_L
  Memory1 : Memory  InitialCondition=T_hs_ini_R_R
  OPEN DIFFERENTIAL EQUATIONS : MATLAB Function  TreatAsAtomicUnit=on
  RIGHT HALF SHAFT TORQUES WITH BACKLASH : Subsystem
  To Workspace : ToWorkspace  VariableName=Tm_RL_sim  SaveFormat=Timeseries  SampleTime=-1
  To Workspace1 : ToWorkspace  VariableName=Tm_RR_sim  SaveFormat=Timeseries  SampleTime=-1
  T_hs_L : Outport
  T_hs_R : Outport  Port=2
  tag scope: Tm_R_L=global, Tm_R_R=global, theta_s_R_L=global, theta_s_R_R=global, theta_s_ddot_R_L=global, theta_s_ddot_R_R=global, theta_s_dot_R_L=global, theta_s_dot_R_R=global
  wires:
  Integrator5/1 -> [theta_s_dot_R_R], RIGHT HALF SHAFT TORQUES WITH BACKLASH/1(omega_s), Integrator3/1  "theta_s_dot_R"
  Integrator4/1 -> [theta_s_dot_R_L], Integrator1/1, LEFT HALF SHAFT TORQUES WITH BACKLASH/1(omega_s)  "theta_s_dot_L"
  Memory1/1 -> OPEN DIFFERENTIAL EQUATIONS/4(T_hs_R)
  Integrator3/1 -> [theta_s_R_R], RIGHT HALF SHAFT TORQUES WITH BACKLASH/2(theta_s)  "theta_s_R"
  theta_w_R/1 -> RIGHT HALF SHAFT TORQUES WITH BACKLASH/3(theta_w)
  omega_w_L/1 -> LEFT HALF SHAFT TORQUES WITH BACKLASH/4(omega_w)
  omega_w_R/1 -> RIGHT HALF SHAFT TORQUES WITH BACKLASH/4(omega_w)
  DIFFERENTIAL_L/1(T_t) -> OPEN DIFFERENTIAL EQUATIONS/1(T_t_L)
  theta_w_L/1 -> LEFT HALF SHAFT TORQUES WITH BACKLASH/3(theta_w)
  Integrator1/1 -> [theta_s_R_L], LEFT HALF SHAFT TORQUES WITH BACKLASH/2(theta_s)  "theta_s_L"
  Memory/1 -> OPEN DIFFERENTIAL EQUATIONS/2(T_hs_L)
  LEFT HALF SHAFT TORQUES WITH BACKLASH/1(T_hs) -> Memory/1, T_hs_L/1  "T_hs_L"
  RIGHT HALF SHAFT TORQUES WITH BACKLASH/1(T_hs) -> T_hs_R/1, Memory1/1  "T_hs_R"
  DIFFERENTIAL_R/1(T_t) -> OPEN DIFFERENTIAL EQUATIONS/3(T_t_R)
  OPEN DIFFERENTIAL EQUATIONS/1(theta_s_ddot_L) -> [theta_s_ddot_R_L], Integrator4/1
  T_m_R/1 -> [Tm_R_R], To Workspace1/1, DIFFERENTIAL_R/1(T_dm)
  T_m_L/1 -> [Tm_R_L], To Workspace/1, DIFFERENTIAL_L/1(T_dm)
  OPEN DIFFERENTIAL EQUATIONS/2(theta_s_ddot_R) -> Integrator5/1, [theta_s_ddot_R_R]

== system Full_Car_Model/PLANT MODEL WITH MF-SWIFT/FRONT LEFT WHEEL ==
  note: Front rotational balance
  Tt_F_L : Inport
  BUS : Inport  Port=2
  Add : Sum
  Bus Creator : BusCreator  Inputs=3
  Bus Selector : BusSelector  OutputSignals=vertical_deflection,effective_rolling_radius,eff_plane_height,eff_plane_angle,Fx,longitudinal_slip,effective_rolling_radius,mu_x
  Clock : Clock
  Constant2 : Constant
  Demux : Demux  Outputs=2
  Gain : Gain  Gain=1/(data.I_y_F)
  Integrate velocity : Integrator  InitialCondition=theta_w_ini_F_L
  Integrate wheel acceleration : Integrator  InitialCondition=omega_ini_F_L
  MF-Swift : mfswift_library/MF-Swift  Tag=STI tyre  idtyre=3  tpfname=tir_name_L  rdfname=[handmade_front,';',handmade_mu_front];  road_mode=(2xxxx) opencrg  side_mode=(x3xxx) symmetric  cnt_mode=(xx5xx) enveloping  dyn_mode=(xxx3x) rigid-ring  mf_mode=(xxxx1) longitudinal  tv_model=Disabled  overwrite=off  use_mode=ISWITCH  internal_solver=off  enable_rr_init=on  optional_input=''  override_typarr=off  disp_debug=off
  Scope : Scope
  "Select Fz, wheel" : Selector  InputPortWidth=3  IndexOptions=Index vector (dialog)  Indices=[1 3]  OutputSizes=[(-2)]
  Select My,wheel : Selector  InputPortWidth=3  IndexOptions=Index vector (dialog)  Indices=2  OutputSizes=[(-2)]
  Subsystem : Subsystem
  Subsystem1 : Subsystem
  Subsystem6 : Subsystem
  Terminator{1..4,12} (5 alike) : Terminator
  To Workspace2 : ToWorkspace  VariableName=force_F_L  SampleTime=-1
  To Workspace3 : ToWorkspace  VariableName=torque_F_L  SampleTime=-1
  local2global : mfswift_library/local2global  Tag=local2global  init_pos=[data.a+data.b 0 (0.3833 - 0.5*data.m_total*9.81*data.b/data.L/data.k_t_F)]  init_angle=[0 0 0]
  Fx_F_L : Outport  VectorParamsAs1DForOutWhenUnconnected=off
  Fz_F_L_tot : Outport  Port=2  VectorParamsAs1DForOutWhenUnconnected=off
  Rotational_F_L : Outport  Port=3  VectorParamsAs1DForOutWhenUnconnected=off
  Slip_F_L : Outport  Port=4  VectorParamsAs1DForOutWhenUnconnected=off
  tag scope: mu_swift_F_L=global, w_swift_F_L=global
  wires:
  Bus Selector/8 -> [mu_swift_F_L], Scope/1  "<mu_x>"
  Bus Creator/1 -> Rotational_F_L/1
  Bus Selector/7 -> Terminator1/1  "<effective_rolling_radius>"
  Bus Selector/6 -> Slip_F_L/1  "<longitudinal_slip>"
  Bus Selector/5 -> Terminator3/1  "<Fx>"
  Bus Selector/2 -> Terminator2/1  "<effective_rolling_radius>"
  Bus Selector/1 -> Terminator12/1  "<vertical_deflection>"
  Bus Selector/3 -> [w_swift_F_L]  "<eff_plane_height>"
  Bus Selector/4 -> Terminator4/1  "<eff_plane_angle>"
  Demux/2 -> Fz_F_L_tot/1  "F_z_F_L"
  Integrate velocity/1 -> MF-Swift/3, Bus Creator/3  "theta_F_L"
  Tt_F_L/1 -> Add/1
  Add/1 -> Gain/1
  local2global/1 -> MF-Swift/1  "r"
  MF-Swift/3 -> Bus Selector/1
  Demux/1 -> Fx_F_L/1  "F_x_F_L"
  "Select Fz, wheel"/1 -> Demux/1
  Clock/1 -> Subsystem6/1(time)
  Subsystem6/1(Road) -> MF-Swift/7  "With enveloping model i don't need this input"
  Constant2/1 -> Subsystem6/2(gain)
  local2global/2 -> MF-Swift/2
  Integrate wheel acceleration/1 -> Integrate velocity/1, MF-Swift/6, Bus Creator/2  "omega_F_L"
  Gain/1 -> Integrate wheel acceleration/1, Bus Creator/1  "omega_dot_F_L"
  MF-Swift/2 -> Select My,wheel/1, To Workspace3/1
  Select My,wheel/1 -> Add/2
  MF-Swift/1 -> "Select Fz, wheel"/1, To Workspace2/1
  Subsystem/1(Velocity) -> local2global/1, MF-Swift/4
  Subsystem1/1(AngularVelocity) -> MF-Swift/5, local2global/2
  BUS/1 -> Subsystem/1(speed), Subsystem1/1(Angular Speed)

== system Full_Car_Model/PLANT MODEL WITH MF-SWIFT/FRONT RIGHT WHEEL ==
  note: Front rotational balance
  Tt_F_R : Inport
  BUS : Inport  Port=2
  Add : Sum
  Bus Creator : BusCreator  Inputs=3
  Bus Selector : BusSelector  OutputSignals=vertical_deflection,effective_rolling_radius,eff_plane_height,eff_plane_angle,Fx,longitudinal_slip,effective_rolling_radius,mu_x
  Clock : Clock
  Constant2 : Constant
  Demux : Demux  Outputs=2
  Gain : Gain  Gain=1/(data.I_y_F)
  Integrate velocity : Integrator  InitialCondition=theta_w_ini_F_L
  Integrate wheel acceleration : Integrator  InitialCondition=omega_ini_F_R
  MF-Swift : mfswift_library/MF-Swift  Tag=STI tyre  idtyre=4  tpfname=tir_name_R  rdfname=[handmade_front,';',handmade_mu_front];  road_mode=(2xxxx) opencrg  side_mode=(x3xxx) symmetric  cnt_mode=(xx5xx) enveloping  dyn_mode=(xxx3x) rigid-ring  mf_mode=(xxxx1) longitudinal  tv_model=Disabled  overwrite=off  use_mode=ISWITCH  internal_solver=off  enable_rr_init=on  optional_input=''  override_typarr=off  disp_debug=off
  "Select Fz, wheel" : Selector  InputPortWidth=3  IndexOptions=Index vector (dialog)  Indices=[1 3]  OutputSizes=[(-2)]
  Select My,wheel : Selector  InputPortWidth=3  IndexOptions=Index vector (dialog)  Indices=2  OutputSizes=[(-2)]
  Subsystem : Subsystem
  Subsystem1 : Subsystem
  Subsystem6 : Subsystem
  Terminator{,1,3..4,12} (5 alike) : Terminator
  To Workspace2 : ToWorkspace  VariableName=force_F_R  SampleTime=-1
  To Workspace3 : ToWorkspace  VariableName=torque_F_R  SampleTime=-1
  local2global : mfswift_library/local2global  Tag=local2global  init_pos=[data.a+data.b 0 (0.3833 - 0.5*data.m_total*9.81*data.b/data.L/data.k_t_F)]  init_angle=[0 0 0]
  Fx_F_R : Outport  VectorParamsAs1DForOutWhenUnconnected=off
  Fz_F_R_tot : Outport  Port=2  VectorParamsAs1DForOutWhenUnconnected=off
  Rotational_F_R : Outport  Port=3  VectorParamsAs1DForOutWhenUnconnected=off
  Slip_F_R : Outport  Port=4  VectorParamsAs1DForOutWhenUnconnected=off
  tag scope: mu_swift_F_R=global, w_swift_F_R=global
  wires:
  Bus Selector/8 -> [mu_swift_F_R]  "<mu_x>"
  Subsystem1/1(AngularVelocity) -> local2global/2, MF-Swift/5
  Subsystem/1(Velocity) -> MF-Swift/4, local2global/1
  MF-Swift/1 -> To Workspace2/1, "Select Fz, wheel"/1
  Select My,wheel/1 -> Add/2
  MF-Swift/2 -> To Workspace3/1, Select My,wheel/1
  Gain/1 -> Bus Creator/1, Integrate wheel acceleration/1  "omega_dot_F_R"
  Integrate wheel acceleration/1 -> Bus Creator/2, MF-Swift/6, Integrate velocity/1  "omega_F_R"
  local2global/2 -> MF-Swift/2
  Constant2/1 -> Subsystem6/2(gain)
  Subsystem6/1(Road) -> MF-Swift/7  "With enveloping model i don't need this input"
  Clock/1 -> Subsystem6/1(time)
  "Select Fz, wheel"/1 -> Demux/1
  Demux/1 -> Fx_F_R/1  "F_x_F_R"
  MF-Swift/3 -> Bus Selector/1
  local2global/1 -> MF-Swift/1  "r"
  Add/1 -> Gain/1
  Tt_F_R/1 -> Add/1
  Integrate velocity/1 -> Bus Creator/3, MF-Swift/3  "theta_F_R"
  Demux/2 -> Fz_F_R_tot/1  "F_z_F"
  Bus Selector/4 -> Terminator4/1  "<eff_plane_angle>"
  Bus Selector/3 -> [w_swift_F_R]  "<eff_plane_height>"
  Bus Selector/1 -> Terminator12/1  "<vertical_deflection>"
  Bus Selector/2 -> Terminator/1  "<effective_rolling_radius>"
  Bus Selector/5 -> Terminator3/1  "<Fx>"
  Bus Selector/6 -> Slip_F_R/1  "<longitudinal_slip>"
  Bus Selector/7 -> Terminator1/1  "<effective_rolling_radius>"
  Bus Creator/1 -> Rotational_F_R/1
  BUS/1 -> Subsystem1/1(Angular Speed), Subsystem/1(speed)

== system Full_Car_Model/PLANT MODEL WITH MF-SWIFT/REAR LEFT WHEEL ==
  note: Rear rotational balance
  Tt_R_L : Inport
  BUS : Inport  Port=2
  Add1 : Sum
  Bus Creator : BusCreator  Inputs=3
  Bus Selector3 : BusSelector  OutputSignals=vertical_deflection,effective_rolling_radius,eff_plane_height,eff_plane_angle,longitudinal_slip,mu_x
  Clock1 : Clock
  Constant3 : Constant
  Demux1 : Demux  Outputs=2
  Gain3 : Gain  Gain=1/(data.I_y_R)
  Integrate velocity1 : Integrator  InitialCondition=theta_w_ini_R_L
  Integrate wheel acceleration : Integrator  InitialCondition=omega_ini_R_L
  MF-Swift : mfswift_library/MF-Swift  Tag=STI tyre  idtyre=1  tpfname=tir_name_L  rdfname=[handmade_rear,';',handmade_mu_rear];  road_mode=(2xxxx) opencrg  side_mode=(x3xxx) symmetric  cnt_mode=(xx5xx) enveloping  dyn_mode=(xxx3x) rigid-ring  mf_mode=(xxxx1) longitudinal  tv_model=Disabled  overwrite=off  use_mode=ISWITCH  internal_solver=off  enable_rr_init=on  optional_input=''  override_typarr=off  disp_debug=off
  "Select Fz, wheel" : Selector  InputPortWidth=3  IndexOptions=Index vector (dialog)  Indices=[1 3]  OutputSizes=[(-2)]
  Select My,wheel1 : Selector  InputPortWidth=3  IndexOptions=Index vector (dialog)  Indices=2  OutputSizes=[(-2)]
  Subsystem2 : Subsystem
  Subsystem5 : Subsystem
  Subsystem7 : Subsystem
  Terminator11 : Terminator
  Terminator13 : Terminator
  Terminator2 : Terminator
  To Workspace1 : ToWorkspace  VariableName=force_R_L  SampleTime=-1
  To Workspace4 : ToWorkspace  VariableName=torque_R_L  SampleTime=-1
  local2global : mfswift_library/local2global  Tag=local2global  init_pos=[0 0 (0.3833 - 0.5*data.m_total*9.81*data.a/data.L/data.k_t_R)]  init_angle=[0 0 0]
  Fx_R_L : Outport  VectorParamsAs1DForOutWhenUnconnected=off
  Fz_R_L_tot : Outport  Port=2  VectorParamsAs1DForOutWhenUnconnected=off
  Rotational_R_L : Outport  Port=3  VectorParamsAs1DForOutWhenUnconnected=off
  Slip_R_L : Outport  Port=4  VectorParamsAs1DForOutWhenUnconnected=off
  tag scope: mu_swift_R_L=global, w_swift_R_L=global
  wires:
  Subsystem5/1(AngularVelocity) -> MF-Swift/5, local2global/2
  BUS/1 -> Subsystem5/1(Angular Speed), Subsystem2/1(speed)
  Select My,wheel1/1 -> Add1/2
  Bus Selector3/3 -> [w_swift_R_L]  "<eff_plane_height>"
  local2global/2 -> MF-Swift/2
  Clock1/1 -> Subsystem7/1(time)
  Bus Selector3/4 -> Terminator11/1  "<eff_plane_angle>"
  Demux1/2 -> Fz_R_L_tot/1
  Bus Selector3/1 -> Terminator13/1  "<vertical_deflection>"
  MF-Swift/3 -> Bus Selector3/1
  MF-Swift/2 -> Select My,wheel1/1, To Workspace4/1
  Subsystem2/1(Velocity) -> MF-Swift/4, local2global/1
  Constant3/1 -> Subsystem7/2(gain)
  MF-Swift/1 -> "Select Fz, wheel"/1, To Workspace1/1
  Bus Selector3/2 -> Terminator2/1  "<effective_rolling_radius>"
  Subsystem7/1(Road) -> MF-Swift/7  "With enveloping model i don't need this input"
  Demux1/1 -> Fx_R_L/1  "Fx_R_L"
  Add1/1 -> Gain3/1
  Tt_R_L/1 -> Add1/1
  "Select Fz, wheel"/1 -> Demux1/1
  local2global/1 -> MF-Swift/1
  Integrate velocity1/1 -> MF-Swift/3, Bus Creator/3  "theta_R_L"
  Bus Creator/1 -> Rotational_R_L/1
  Integrate wheel acceleration/1 -> MF-Swift/6, Bus Creator/2, Integrate velocity1/1  "omega_R_L"
  Gain3/1 -> Bus Creator/1, Integrate wheel acceleration/1  "omega_dot_R_L"
  Bus Selector3/5 -> Slip_R_L/1  "<longitudinal_slip>"
  Bus Selector3/6 -> [mu_swift_R_L]  "<mu_x>"
